simulink model "state_space_1"  (Simulink 5.0)
settings: Solver=ode45  StartTime=0.0  StopTime=10.0  RelTol=1e-3
values from neighbouring files (symbols this model uses):
  A = [0,                     0,  1/R,    0,          0,  0,  0,  Vn/R^2,         0 ... (first row only)    [Ainit.m]    (also in coupled_osc.m = [       0                 1             0           0; matlab_demo.m = [1 2 3; 4 5 6; 7 8 9])
  B = zeros(9,9)    [Ainit.m]    (also in coupled_osc.m = [0 0 0 0]'; matlab_demo.m = inv(A))
  C = eye(9)    [Ainit.m]    (also in coupled_osc.m = [1 0 0 0; matlab_demo.m = A')
  D = zeros(9,9)    [Ainit.m]    (also in compute_ud.m = []; coupled_osc.m = [0; matlab_demo.m = u*u')
libraries: simulink x1
settings Model: Creator=mcarroll  LastModifiedBy=mcarroll  ExtModeAutoUpdateStatusClock=off

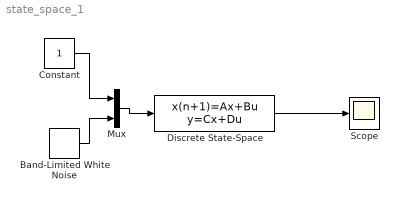
== system state_space_1 ==
  Band-Limited White Noise : simulink/Sources/Band-Limited White Noise  Cov=[0.1]  Ts=0.1  seed=[23341]
  Constant : Constant
  Discrete State-Space : DiscreteStateSpace  A=A  B=B  C=C  D=D
  Mux : Mux  Inputs=2
  Scope : Scope
  wires:
  Discrete State-Space/1 -> Scope/1
  Band-Limited White Noise/1 -> Mux/2
  Constant/1 -> Mux/1
  Mux/1 -> Discrete State-Space/1
